simulink model "UAM_Hexa_PD_Obs"  (R2026b)
settings: Solver=ode4  StopTime=80  FixedStep=0.01
undefined symbols (not defined in the file): ArmConstants, HexaConstants, Observer, PID
libraries: simulink x8
settings Model: Creator=Carlos Fabian  LastModifiedBy=cfmm
settings SimscapeCC: SimscapeLogType=all  SimscapeNominalValues="[{\"value\":\"1\",\"unit\":\"A\"},{\"value\":\"1\",\"unit\":\"bar\"},{\"value\":\"1\",\"unit\":\"cm^2\"},{\"value\":\"1\",\"unit\":\"cm^3/s\"},{\"value\":\"1\",\"unit\":\"kJ/kg\"},{\"value\":\"1\",\"unit\":\"kW\"},{\"value\":\"1\",\"unit\":\"l\"},{\"value\":\"1\",\"unit\":\"N\"},{\"value\":\"1\",\"unit\":\"N*m\"},{\"value\":\"1\",\"unit\":\"V\"},{\"value\":\"0.001\",\"unit\":\"Wb\"}]"  SimscapeUseEnergyAccounting=off
settings ExplorerConfigSet: InternalSimMechanicsExplorerSettings=|
  | <ExplorerConfiguration>
  | 
  |   <canonicalview>default</canonicalview>
  | 
  |   <TilePanel>
  |     <TileInfo>
  |       <Tiles Columns="1" Count="1" Height="826" Rows="1" Width="1394">
  |         <Row Weight="1"/>
  |         <Column Weight="1"/>
  |         <Tile Height="1" Width="1" X="0" Y="0"/>
  |       </Tiles>
  |     </TileInfo>
  |     <SceneInfo>
  |       <SceneViewer>
  |         <IsThisViewStd>
  |           <IsStandardView>off</IsStandardView>
  |           <StandardViewName>Front</StandardViewName>
  |         </IsThisViewStd>
  |         <BGColor>
  |           <R>1</R>
  |           <G>1</G>
  |           <B>1</B>
  |           <A>1</A>
  |         </BGColor>
  |         <Camera>
  |           <DoPerspective>off</DoPerspective>
  |           <Position>
  |             <X>0</X>
  |             <Y>-34.647213736646918</Y>
  |             <Z>3.330955067047817</Z>
  |           </Position>
  |           <Center>
  |             <X>0</X>
  |             <Y>0</Y>
  |             <Z>3.330955067047817</Z>
  |           </Center>
  |           <Up>
  |             <X>0</X>
  |             <Y>0</Y>
  |             <Z>1</Z>
  |           </Up>
  |           <XLim>3.4308837190592514</XLim>
  |           <YLim>3.4308837190592514</YLim>
  |           <ViewLimDist>0.01</ViewLimDist>
  |         </Camera>
  |       </SceneViewer>
  |     </SceneInfo>
  |   </TilePanel>
  | 
  |   <MechEditorPanel>
  |     <GfxPanelCameraMap/>
  |     <Cameras/>
  |     <VideoCreator>
  |       <IncludeTiles>All</IncludeTiles>
  |       <IncludeTime>on</IncludeTime>
  |       <IncludeWorldFrame>off</IncludeWorldFrame>
  |       <PlaybackSpeedRatio>8</PlaybackSpeedRatio>
  |       <FrameRate>24</FrameRate>
  |       <FrameSize>auto</FrameSize>
  |       <VideoFormat>MotionJPEGAVI</VideoFormat>
  |     </VideoCreator>
  |   </MechEditorPanel>
  | 
  |   <PlaybackSettings>
  |     <PlaybackSpeedFactor>1</PlaybackSpeedFactor>
  |   </PlaybackSettings>
  | 
  | </ExplorerConfiguration>

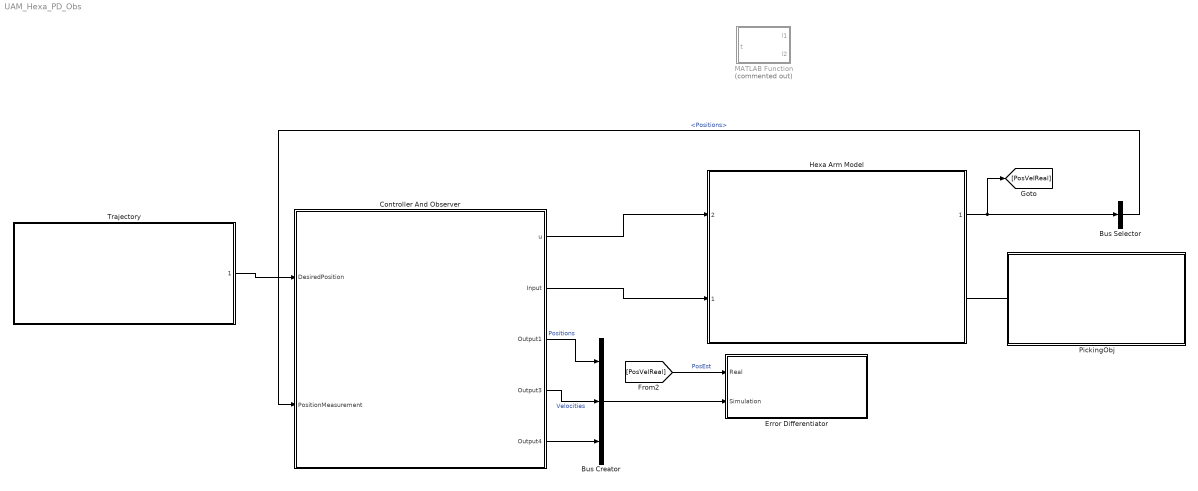
== system UAM_Hexa_PD_Obs ==
  Bus Creator : BusCreator  Inputs=3
  Bus Selector : BusSelector  OutputSignals=Positions
  Controller And Observer : Subsystem
  Error Differentiator : Subsystem
  Hexa Arm Model : Subsystem  ReferencedSubsystem=HexaArmModel
      settings: PortSchema="{\"entries\":[{\"content\":{\"sides\":[{\"content\":{\"connectorIds\":[\"In2\",\"In1\"]},\"type\":\"ConnectorPlacement.EquallySpacedRectSide\",\"uuid\":\"8c321911-c61a-4c60-b031-eeaf4c8b5083\"},{\"content\":{\"connectorIds\":[\"Out1\",\"RConn1\"],\"side\":\"RIGHT\"},\"type\":\"ConnectorPlacement.EquallySpacedRectSide\",\"uuid\":\"3ad1588f-e2f8-4666-8b86-318f5207193d\"},{\"content\":{\"side\":\"TOP\"},\"type\":\"ConnectorPlacement.EquallySpacedRectSide\",\"uuid\":\"710cc49c-59c4-4f69-a558-4588d1d119c0\"}]},\"type\":\"ConnectorPlacement.EquallySpacedConnector\",\"uuid\":\"3e8cca1f-f7f1-4f31-9eba-ef93ff8e81e8\"}],\"packageUris\":[\"http://schema.mathworks.com/mf0/Connector/R2020b\"],\"version\":\"1.0\"}"
  MATLAB Function : MATLAB Function  Commented=on  TreatAsAtomicUnit=on
  PickingObj : Subsystem  ReferencedSubsystem=PickingObj
  Trajectory : Subsystem  ReferencedSubsystem=TrajectoryGeneration
  wires:
  Controller And Observer/2(Input) -> Hexa Arm Model/1
  Trajectory/1 -> Controller And Observer/1(DesiredPosition)
  Hexa Arm Model/1 -> [PosVelReal], Bus Selector/1
  Controller And Observer/1(u) -> Hexa Arm Model/2
  Bus Selector/1 -> Controller And Observer/2(PositionMeasurement)  "<Positions>"
  [PosVelReal] -> Error Differentiator/1(Real)  "PosEst"
  Controller And Observer/4(Output3) -> Bus Creator/2  "Velocities"
  Controller And Observer/3(Output1) -> Bus Creator/1  "Positions"
  Bus Creator/1 -> Error Differentiator/2(Simulation)
  Controller And Observer/5(Output4) -> Bus Creator/3
  connections:
  Hexa Arm Model/RConn1 -- PickingObj/LConn1

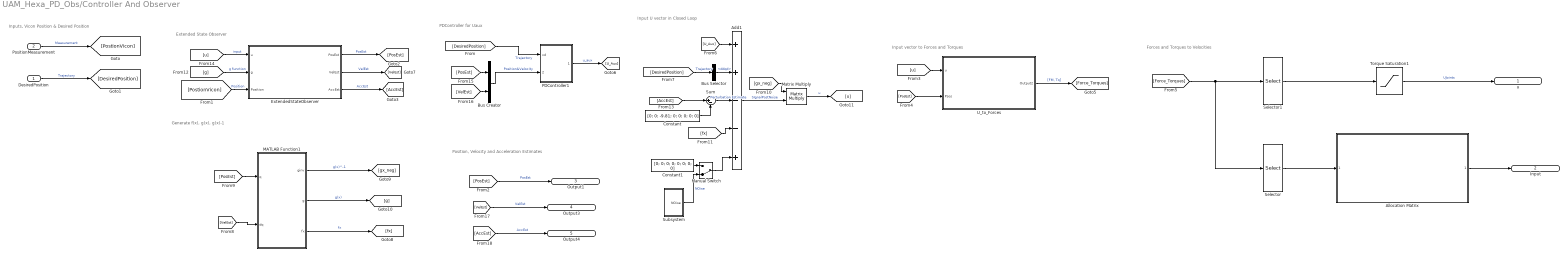
== system UAM_Hexa_PD_Obs/Controller And Observer ==
  note: Position, Velocity and Acceleration Estimates
  note: Input vector to Forces and Torques
  note: Forces and Torques to Velocities
  note: Extended State Observer
  note: Input U vector in Closed Loop
  note: Generate f(x), g(x), g(x)-1
  note: PDController for Uaux
  note: Inputs, Vicon Position & Desired Position
  DesiredPosition : Inport
  PositionMeasurement : Inport  Port=2
  Add1 : Sum  Inputs=++--+
  Allocation Matrix : Subsystem  ReferencedSubsystem=FromFMtoOmega2
  Bus Creator : BusCreator  Inputs=2
  Bus Selector : BusSelector  OutputSignals=ddqd
  Constant : Constant  Value=[0; 0; -9.81; 0; 0; 0; 0; 0]
  Constant1 : Constant  Value=[0; 0; 0; 0; 0; 0; 0; 0]
  ExtendedStateObserver : Subsystem
  MATLAB Function1 : MATLAB Function  TreatAsAtomicUnit=on
  Manual Switch : ManualSwitch  CurrentSetting=0
  Matrix Multiply : Product  Multiplication=Matrix(*)
  PDController1 : Subsystem
  Selector : Selector  InputPortWidth=8  IndexOptions=Index vector (dialog)  Indices=1:6  OutputSizes=1  RuntimeRangeChecks=off
  Selector1 : Selector  InputPortWidth=8  IndexOptions=Index vector (dialog)  Indices=7:8  OutputSizes=1  RuntimeRangeChecks=off
  Subsystem : Subsystem
  Sum : Sum  Inputs=|+-
  Torque Saturation1 : Saturate  UpperLimit=ArmConstants.Servos.T1max  LowerLimit=-ArmConstants.Servos.T1max
  U_to_Forces : Subsystem
  u : Outport
  Input : Outport  Port=2
  Output1 : Outport  Port=3
  Output3 : Outport  Port=4
  Output4 : Outport  Port=5
  wires:
  [PostionVicon] -> ExtendedStateObserver/3(Position)  "Position"
  [DesiredPosition] -> PDController1/1(xd)  "Trajectory"
  U_to_Forces/1(Output2) -> [Force_Torques]  "[FM, Tq]"
  ExtendedStateObserver/1(PosEst) -> [PosEst]  "PosEst"
  PositionMeasurement/1 -> [PostionVicon]  "Measurement"
  DesiredPosition/1 -> [DesiredPosition]  "Trajectory"
  Bus Creator/1 -> PDController1/2(q_hat1)  "Position&Velocity"
  ExtendedStateObserver/3(AccEst) -> [AccEst]  "AccEst"
  ExtendedStateObserver/2(VelEst) -> [VelEst]  "VelEst"
  [PosEst] -> U_to_Forces/2(Psos)
  Selector1/1 -> Torque Saturation1/1
  [Force_Torques] -> Selector/1, Selector1/1
  Selector/1 -> Allocation Matrix/1
  Torque Saturation1/1 -> u/1  "UJoints"
  Allocation Matrix/1 -> Input/1
  PDController1/1(Output) -> [U_Aux]  "u_aux"
  MATLAB Function1/1(ginv) -> [gx_neg]  "g(x)^-1"
  MATLAB Function1/3(fx) -> [fx]  "fx"
  [VelEst] -> MATLAB Function1/2(dq)
  [PosEst] -> MATLAB Function1/1(q)
  [fx] -> Add1/4
  Add1/1 -> Matrix Multiply/2  "SIgnalPostNoise"
  Matrix Multiply/1 -> [u]  "u"
  [gx_neg] -> Matrix Multiply/1
  [U_Aux] -> Add1/1
  [DesiredPosition] -> Bus Selector/1  "Trajectory"
  Bus Selector/1 -> Add1/2  "<ddqd>"
  [AccEst] -> Sum/1
  MATLAB Function1/2(g) -> [g]  "g(x)"
  [g] -> ExtendedStateObserver/2(g)  "g function"
  [u] -> ExtendedStateObserver/1(u)  "input"
  [PosEst] -> Bus Creator/1
  [VelEst] -> Bus Creator/2
  [u] -> U_to_Forces/1(u)
  [PosEst] -> Output1/1  "PosEst"
  [VelEst] -> Output3/1  "VelEst"
  [AccEst] -> Output4/1  "AccEst"
  Sum/1 -> Add1/3  "Perturbation Estimate"
  Constant/1 -> Sum/2
  Subsystem/1(NOise) -> Manual Switch/2  "NOise"
  Manual Switch/1 -> Add1/5
  Constant1/1 -> Manual Switch/1

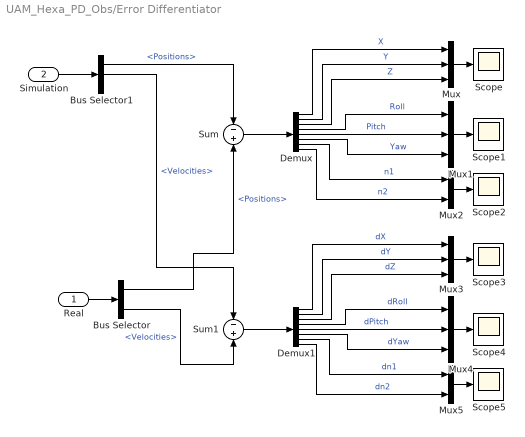
== system UAM_Hexa_PD_Obs/Error Differentiator ==
  Real : Inport
  Simulation : Inport  Port=2
  Bus Selector : BusSelector  OutputSignals=Positions,Velocities
  Bus Selector1 : BusSelector  OutputSignals=Positions,Velocities,AccEst
  Demux : Demux  Outputs=8
  Demux1 : Demux  Outputs=8
  Mux{,1,3..4} (4 alike) : Mux  Inputs=3
  Mux2 : Mux  Inputs=2
  Mux5 : Mux  Inputs=2
  Scope{,1..5} (6 alike) : Scope
      Scope settings: ActiveDisplayYMinimum=-0.12805242657923774  ActiveDisplayYMaximum=0.1215294954009426
      Scope1 settings: ActiveDisplayYMinimum=-0.0054009288599574049  ActiveDisplayYMaximum=0.0052845116621625422  DataLoggingVariableName=ScopeData4
      Scope2 settings: ActiveDisplayYMinimum=-0.10904794631046834  ActiveDisplayYMaximum=0.0987033920807902  DataLoggingVariableName=ScopeData5
      Scope3 settings: ActiveDisplayYMinimum=-0.012418640162776391  ActiveDisplayYMaximum=0.059212364522656324  DataLoggingVariableName=ScopeData6
      Scope4 settings: ActiveDisplayYMinimum=-0.047205139628020171  ActiveDisplayYMaximum=0.05488863646197175  DataLoggingVariableName=ScopeData7
      Scope5 settings: ActiveDisplayYMinimum=-6.6425457150387848  ActiveDisplayYMaximum=5.5018292085843479  DataLoggingVariableName=ScopeData8
  Sum : Sum  Inputs=-+
  Sum1 : Sum  Inputs=-+
  wires:
  Mux2/1 -> Scope2/1
  Sum/1 -> Demux/1
  Mux1/1 -> Scope1/1
  Bus Selector1/1 -> Sum/1  "<Positions>"
  Demux/8 -> Mux2/2  "n2"
  Bus Selector/2 -> Sum1/2  "<Velocities>"
  Demux/7 -> Mux2/1  "n1"
  Mux/1 -> Scope/1
  Demux/1 -> Mux/1  "X"
  Demux/4 -> Mux1/1  "Roll"
  Demux/6 -> Mux1/3  "Yaw"
  Demux/5 -> Mux1/2  "Pitch"
  Demux/3 -> Mux/3  "Z"
  Bus Selector/1 -> Sum/2  "<Positions>"
  Demux/2 -> Mux/2  "Y"
  Bus Selector1/2 -> Sum1/1  "<Velocities>"
  Simulation/1 -> Bus Selector1/1
  Real/1 -> Bus Selector/1
  Demux1/8 -> Mux5/2  "dn2"
  Mux4/1 -> Scope4/1
  Sum1/1 -> Demux1/1
  Mux5/1 -> Scope5/1
  Demux1/4 -> Mux4/1  "dRoll"
  Demux1/6 -> Mux4/3  "dYaw"
  Demux1/2 -> Mux3/2  "dY"
  Demux1/1 -> Mux3/1  "dX"
  Mux3/1 -> Scope3/1
  Demux1/5 -> Mux4/2  "dPitch"
  Demux1/7 -> Mux5/1  "dn1"
  Demux1/3 -> Mux3/3  "dZ"

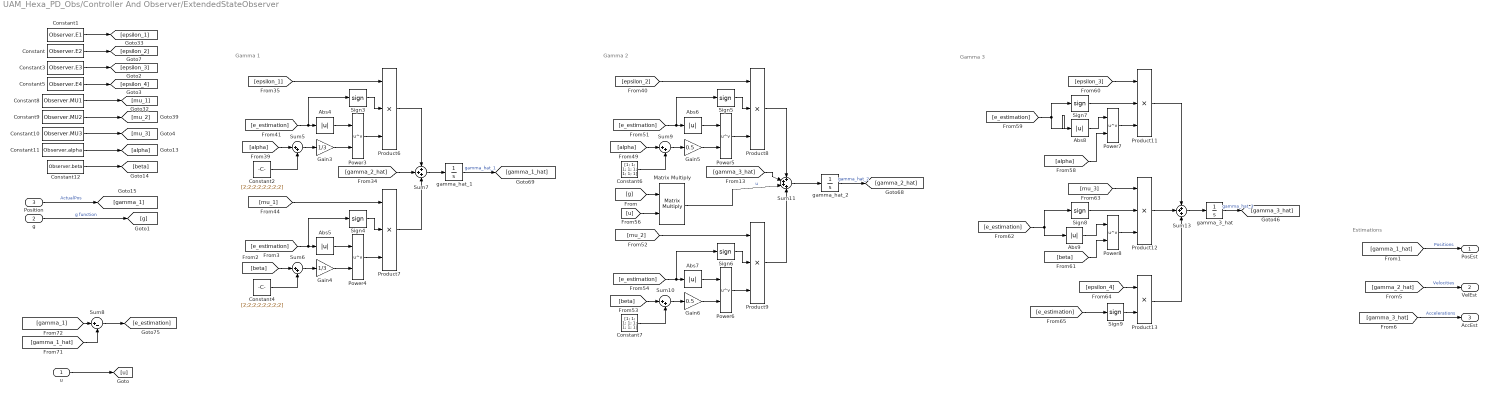
== system UAM_Hexa_PD_Obs/Controller And Observer/ExtendedStateObserver ==
  note: Estimations
  note: Gamma 3
  note: Gamma 2
  note: Gamma 1
  u : Inport
  g : Inport  Port=2
  Position : Inport  Port=3
  Abs{4..9} (6 alike) : Abs  SaturateOnIntegerOverflow=off
  Constant : Constant  Value=Observer.E2
  Constant1 : Constant  Value=Observer.E1
  Constant10 : Constant  Value=Observer.MU3
  Constant11 : Constant  Value=Observer.alpha
  Constant12 : Constant  Value=Observer.beta
  Constant2 : Constant  Value=[2;2;2;2;2;2;2;2]
  Constant3 : Constant  Value=Observer.E3
  Constant4 : Constant  Value=[2;2;2;2;2;2;2;2]
  Constant5 : Constant  Value=Observer.E4
  Constant6 : Constant  Value=[1; 1; 1; 1; 1; 1; 1; 1]
  Constant7 : Constant  Value=[1; 1; 1; 1; 1; 1; 1; 1]
  Constant8 : Constant  Value=Observer.MU1
  Constant9 : Constant  Value=Observer.MU2
  Gain3 : Gain  Gain=1/3
  Gain4 : Gain  Gain=1/3
  Gain5 : Gain  Gain=0.5
  Gain6 : Gain  Gain=0.5
  Matrix Multiply : Product  Multiplication=Matrix(*)
  Power{3..8} (6 alike) : Math  Operator=pow
  Product{6..9,11..12} (6 alike) : Product  Inputs=3
  Product13 : Product
  Sign{3..9} (7 alike) : Signum
  Sum{5..6,9..10} (4 alike) : Sum  Inputs=|++
  Sum11 : Sum  Inputs=++++
  Sum13 : Sum  Inputs=+++
  Sum7 : Sum  Inputs=+++
  Sum8 : Sum  Inputs=|+-
  gamma_3_hat : Integrator  InitialCondition=[0; 0; -9.81; 0; 0; 0; 0; 0]
  gamma_hat_1 : Integrator  InitialCondition=[0; 0; 0.24; 0; 0; 0; 0; 0]
  gamma_hat_2 : Integrator  InitialCondition=zeros(8,1)
  PosEst : Outport
  VelEst : Outport  Port=2
  AccEst : Outport  Port=3
  wires:
  Constant11/1 -> [alpha]
  [beta] -> Sum10/1
  [e_estimation] -> Sign8/1, Abs9/1
  Power7/1 -> Product11/3
  Matrix Multiply/1 -> Sum11/3  "u"
  Constant12/1 -> [beta]
  [e_estimation] -> Abs8/1, Sign7/1
  [gamma_1_hat] -> PosEst/1  "Positions"
  Power8/1 -> Product12/3
  Constant4/1 -> Sum6/2
  [alpha] -> Sum5/1
  Product6/1 -> Sum7/1
  Abs8/1 -> Power7/1
  Power5/1 -> Product8/3
  [gamma_1] -> Sum8/1
  [e_estimation] -> Sign6/1, Abs7/1
  [epsilon_2] -> Product8/1
  Sum11/1 -> gamma_hat_2/1
  Constant10/1 -> [mu_3]
  Gain5/1 -> Power5/2
  [e_estimation] -> Sign3/1, Abs4/1
  Abs5/1 -> Power4/1
  Sum13/1 -> gamma_3_hat/1
  Abs7/1 -> Power6/1
  Product9/1 -> Sum11/4
  [epsilon_1] -> Product6/1
  Constant7/1 -> Sum10/2
  [epsilon_3] -> Product11/1
  Sum9/1 -> Gain5/1
  Sum6/1 -> Gain4/1
  [e_estimation] -> Sign5/1, Abs6/1
  u/1 -> [u]
  [mu_3] -> Product12/1
  Sign6/1 -> Product9/2
  Sum7/1 -> gamma_hat_1/1
  Sign8/1 -> Product12/2
  [alpha] -> Power7/2
  [epsilon_4] -> Product13/1
  [gamma_3_hat] -> Sum11/2
  [mu_1] -> Product7/1
  Sign3/1 -> Product6/2
  gamma_hat_2/1 -> [gamma_2_hat]  "gamma_hat_2"
  Constant/1 -> [epsilon_2]
  [mu_2] -> Product9/1
  Product11/1 -> Sum13/1
  [gamma_1_hat] -> Sum8/2
  Sign4/1 -> Product7/2
  Product7/1 -> Sum7/3
  Constant9/1 -> [mu_2]
  Constant1/1 -> [epsilon_1]
  Constant6/1 -> Sum9/2
  Sign5/1 -> Product8/2
  [beta] -> Power8/2
  Constant2/1 -> Sum5/2
  Gain6/1 -> Power6/2
  Gain3/1 -> Power3/2
  Power6/1 -> Product9/3
  Position/1 -> [gamma_1]  "ActualPos"
  Constant5/1 -> [epsilon_4]
  Constant3/1 -> [epsilon_3]
  Product13/1 -> Sum13/3
  gamma_hat_1/1 -> [gamma_1_hat]  "gamma_hat_1"
  Sum5/1 -> Gain3/1
  Power3/1 -> Product6/3
  Power4/1 -> Product7/3
  Sum10/1 -> Gain6/1
  [gamma_2_hat] -> Sum7/2
  Sign7/1 -> Product11/2
  [beta] -> Sum6/1
  [e_estimation] -> Sign4/1, Abs5/1
  [e_estimation] -> Sign9/1
  Product8/1 -> Sum11/1
  Sign9/1 -> Product13/2
  Abs9/1 -> Power8/1
  [alpha] -> Sum9/1
  gamma_3_hat/1 -> [gamma_3_hat]  "gamma_hat_3"
  Sum8/1 -> [e_estimation]
  Gain4/1 -> Power4/2
  Constant8/1 -> [mu_1]
  Product12/1 -> Sum13/2
  g/1 -> [g]  "g function"
  Abs6/1 -> Power5/1
  Abs4/1 -> Power3/1
  [gamma_3_hat] -> AccEst/1  "Accelerations"
  [gamma_2_hat] -> VelEst/1  "Velocities"
  [g] -> Matrix Multiply/1
  [u] -> Matrix Multiply/2

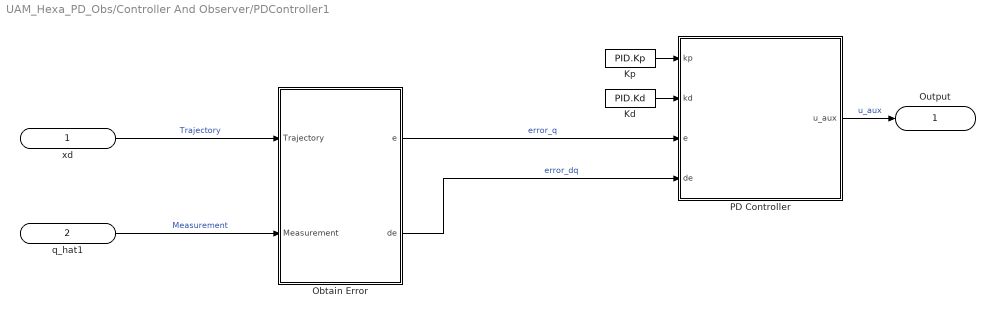
== system UAM_Hexa_PD_Obs/Controller And Observer/PDController1 ==
  xd : Inport
  q_hat1 : Inport  Port=2
  Kd : Constant  Value=PID.Kd
  Kp : Constant  Value=PID.Kp
  Obtain Error : Subsystem
  PD Controller : MATLAB Function  TreatAsAtomicUnit=on
  Output : Outport
  wires:
  xd/1 -> Obtain Error/1(Trajectory)  "Trajectory"
  q_hat1/1 -> Obtain Error/2(Measurement)  "Measurement"
  Obtain Error/1(e) -> PD Controller/3(e)  "error_q"
  Obtain Error/2(de) -> PD Controller/4(de)  "error_dq"
  Kp/1 -> PD Controller/1(kp)
  Kd/1 -> PD Controller/2(kd)
  PD Controller/1(u_aux) -> Output/1  "u_aux"

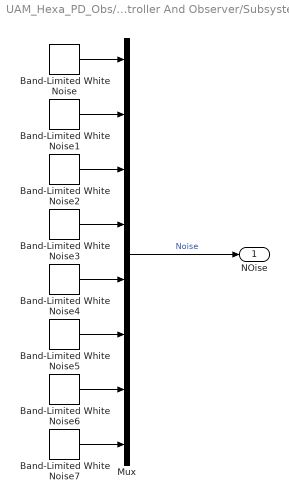
== system UAM_Hexa_PD_Obs/Controller And Observer/Subsystem ==
  Band-Limited White Noise : simulink/Sources/Band-Limited White Noise  Cov=[0.0000001]  Ts=0.01  seed=[23341]
  Band-Limited White Noise1 : simulink/Sources/Band-Limited White Noise  Cov=[0.0000001]  Ts=0.01  seed=[23341]
  Band-Limited White Noise2 : simulink/Sources/Band-Limited White Noise  Cov=[0.000001]  Ts=0.01  seed=[23341]
  Band-Limited White Noise3 : simulink/Sources/Band-Limited White Noise  Cov=[0.000001]  Ts=0.01  seed=[23341]
  Band-Limited White Noise4 : simulink/Sources/Band-Limited White Noise  Cov=[0.000001]  Ts=0.01  seed=[23341]
  Band-Limited White Noise5 : simulink/Sources/Band-Limited White Noise  Cov=[0.0000001]  Ts=0.01  seed=[23341]
  Band-Limited White Noise6 : simulink/Sources/Band-Limited White Noise  Cov=[0.01]  Ts=0.01  seed=[23341]
  Band-Limited White Noise7 : simulink/Sources/Band-Limited White Noise  Cov=[0.02]  Ts=0.01  seed=[23341]
  Mux : Mux  Inputs=8
  NOise : Outport
  wires:
  Mux/1 -> NOise/1  "Noise"
  Band-Limited White Noise/1 -> Mux/1
  Band-Limited White Noise1/1 -> Mux/2
  Band-Limited White Noise2/1 -> Mux/3
  Band-Limited White Noise3/1 -> Mux/4
  Band-Limited White Noise4/1 -> Mux/5
  Band-Limited White Noise5/1 -> Mux/6
  Band-Limited White Noise6/1 -> Mux/7
  Band-Limited White Noise7/1 -> Mux/8

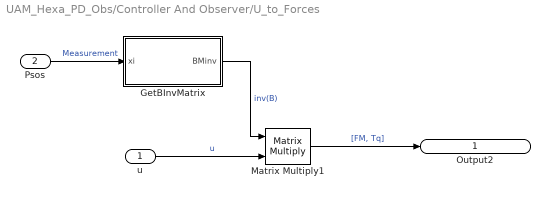
== system UAM_Hexa_PD_Obs/Controller And Observer/U_to_Forces ==
  u : Inport
  Psos : Inport  Port=2
  GetBInvMatrix : MATLAB Function  TreatAsAtomicUnit=on
  Matrix Multiply1 : Product  Multiplication=Matrix(*)
  Output2 : Outport
  wires:
  Psos/1 -> GetBInvMatrix/1(xi)  "Measurement"
  u/1 -> Matrix Multiply1/2  "u"
  Matrix Multiply1/1 -> Output2/1  "[FM, Tq]"
  GetBInvMatrix/1(BMinv) -> Matrix Multiply1/1  "inv(B)"

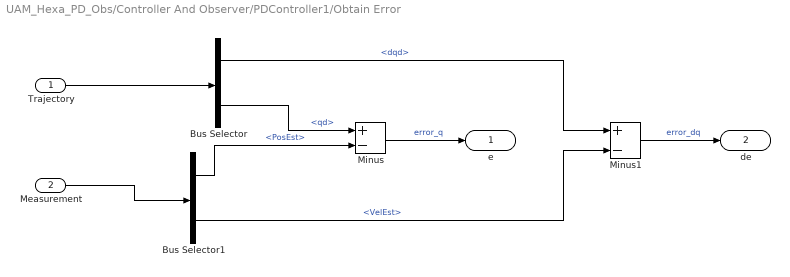
== system UAM_Hexa_PD_Obs/Controller And Observer/PDController1/Obtain Error ==
  Trajectory : Inport
  Measurement : Inport  Port=2
  Bus Selector : BusSelector  OutputSignals=dqd,qd
  Bus Selector1 : BusSelector  OutputSignals=PosEst,VelEst
  Minus : Sum  Inputs=+-
  Minus1 : Sum  Inputs=+-
  e : Outport
  de : Outport  Port=2
  wires:
  Bus Selector1/1 -> Minus/2  "<PosEst>"
  Bus Selector1/2 -> Minus1/2  "<VelEst>"
  Measurement/1 -> Bus Selector1/1
  Trajectory/1 -> Bus Selector/1
  Bus Selector/1 -> Minus1/1  "<dqd>"
  Bus Selector/2 -> Minus/1  "<qd>"
  Minus/1 -> e/1  "error_q"
  Minus1/1 -> de/1  "error_dq"

== matlab function UAM_Hexa_PD_Obs/Controller And Observer/PDController1/PD Controller ==
  data: kp input; kd input; u_aux output; e input; de input
function u_aux = pd_cont(kp, kd, e, de)


kp_m = [kp(1) 0       0     0     0       0     0     0;
        0     kp(2)   0     0     0       0     0     0;
        0     0       kp(3) 0     0       0     0     0;
        0     0       0     kp(4) 0       0     0     0;
        0     0       0     0     kp(5)   0     0     0;
        0     0       0     0     0       kp(6) 0     0;
        0     0       0     0     0       0     kp(7) 0;
        0     0       0     0     0       0     0     kp(8)];

kd_m = [kd(1) 0       0     0     0       0     0     0;
        0     kd(2)   0     0     0       0     0     0;
        0     0       kd(3) 0     0       0     0     0;
        0     0       0     kd(4) 0       0     0     0;
        0     0       0     0     kd(5)   0     0     0;
        0     0       0     0     0       kd(6) 0     0;
        0     0       0     0     0       0     kd(7) 0;
        0     0       0     0     0       0     0     kd(8)];


%v = ddP + kp_m * e + kd_m * de;
u_aux = kp_m * e + kd_m * de;
%v = ddP;

end

== matlab function UAM_Hexa_PD_Obs/MATLAB Function ==
  data: t input; l1 output; l2 output
function [l1, l2] = fcn(t)
t1 = t(1);
t2 = t(2);
i1 = diag([0.00005484, 0.00050874,  0.00046501]);
i2 = diag([0.00008085, 0.00034964,  0.00030340]);

== matlab function UAM_Hexa_PD_Obs/Controller And Observer/MATLAB Function1 ==
  data: q input; dq input; HexaConstants parameter; ginv output; g output; fx output; ArmConstants parameter
function [ginv, g, fx] = Get_DCG_Hexa(q, dq, HexaConstants, ArmConstants)

DM = DMatrix(q, HexaConstants, ArmConstants);
CM = CMatrix(q, dq, HexaConstants, ArmConstants);
Gv = GVector(q, HexaConstants, ArmConstants);

g = inv(DM);
ginv = DM;

fx = DM\( -CM*dq - Gv );

end

== matlab function UAM_Hexa_PD_Obs/Controller And Observer/U_to_Forces/GetBInvMatrix ==
  data: xi input; BMinv output
function BMinv = GetBInvMatrix(xi)

% phi = xi(4);
% th  = xi(5);
% psi = xi(6);
% 
% BM1=[cos(phi)*cos(th),-cos(phi)*sin(psi)+cos(psi)*sin(phi)*sin(th), ...
%     sin(phi)*sin(psi)+cos(phi)*cos(psi)*sin(th),0,0,0;...
%     cos(th)*sin(psi), cos(phi)*cos(psi)+sin(phi)*sin(psi)*sin(th),...
%     -cos(psi)*sin(phi)+cos(phi)*sin(psi)*sin(phi),0,0,0;...
%     -sin(th),cos(th)*sin(psi),cos(phi)*cos(th),0,0,0;...
%     0,0,0,1,sin(phi)*tan(th),cos(phi)*tan(th);...
%     0,0,0,0,cos(phi),-sin(phi);0,0,0,0,sec(th)*sin(phi),cos(phi)*sec(th)];

BM1 = BMatrix(xi);

BM = blkdiag(BM1, eye(2,2));

BMinv = inv(BM);

end
